simulink model "backtoback_harness"  (R2026b)
settings: Solver=ode4  StopTime=8  FixedStep=0.001
undefined symbols (not defined in the file or in its folder): Dgainphi, Igainphi, Pgainphi, ref_phi
libraries: slpidlib x1
settings Model: Creator=Minh  LastModifiedBy=Minh
settings DataIOCC: SaveTime=off

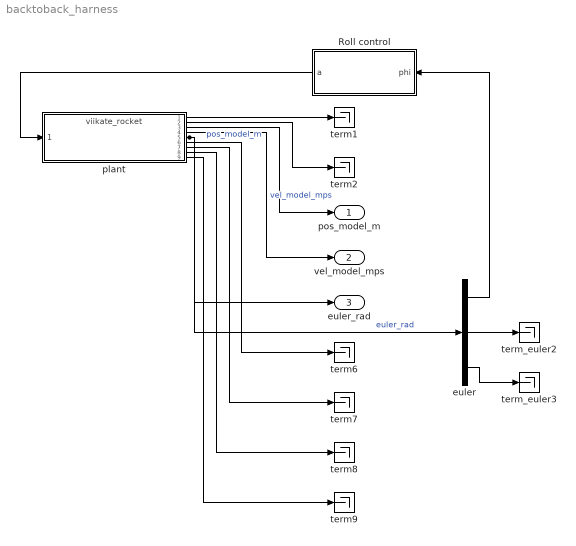
== system backtoback_harness ==
  Roll control : Subsystem
  euler : Demux  Outputs=3
  plant : ModelReference  ModelNameDialog=viikate_rocket  SimulationMode=Normal  ModelReferenceVersion=5.1
  term{1..2,6..9} (6 alike) : Terminator
  term_euler2 : Terminator
  term_euler3 : Terminator
  pos_model_m : Outport
  vel_model_mps : Outport  Port=2
  euler_rad : Outport  Port=3
  wires:
  euler/3 -> term_euler3/1
  euler/2 -> term_euler2/1
  euler/1 -> Roll control/1(phi)
  Roll control/1(a) -> plant/1
  plant/9 -> term9/1
  plant/8 -> term8/1
  plant/7 -> term7/1
  plant/5 -> euler_rad/1, euler/1  "euler_rad"
  plant/4 -> vel_model_mps/1  "vel_model_mps"
  plant/3 -> pos_model_m/1  "pos_model_m"
  plant/6 -> term6/1
  plant/2 -> term2/1
  plant/1 -> term1/1

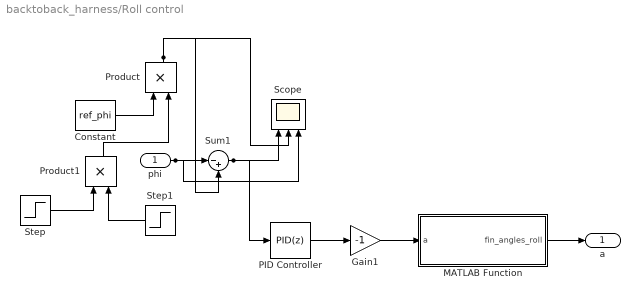
== system backtoback_harness/Roll control ==
  phi : Inport
  Constant : Constant  Value=ref_phi
  Gain1 : Gain  Gain=-1
  MATLAB Function : MATLAB Function  TreatAsAtomicUnit=on
  PID Controller : slpidlib/PID Controller  Controller=PID  Form=Parallel  TimeDomain=Discrete-time  UseExternalTs=off  SampleTime=0.001  IntegratorMethod=Forward Euler  FilterMethod=Forward Euler  ControllerParametersSource=internal  P=Pgainphi  I=Igainphi  UseKiTs=off  D=Dgainphi  UseExternalDerivativeSource=off  N=100  UseFilter=off  TunerSelectOption=Transfer Function Based (PID Tuner App)  InitialConditionSource=internal  InitialConditionForIntegrator=0  InitialConditionForFilter=0  DifferentiatorICPrevScaledInput=0  ExternalReset=none  TrackingMode=off  Kt=1  LimitOutput=on  SatLimitsSource=internal  UpperSaturationLimit=deg2rad(20)  LowerSaturationLimit=-deg2rad(20)  LinearizeAsGain=on  AntiWindupMode=clamping  Kb=1  LimitIntegrator=on  UpperIntegratorSaturationLimit=deg2rad(20)  LowerIntegratorSaturationLimit=-deg2rad(20)  POutMin=[]  POutMax=[]  IOutMin=[]  IOutMax=[]  DOutMin=[]  DOutMax=[]  NOutMin=[]  NOutMax=[]  SumOutMin=[]  SumOutMax=[]  SaturationOutMin=[]  SaturationOutMax=[]  PParamMin=[]  PParamMax=[]  IParamMin=[]  IParamMax=[]  DParamMin=[]  DParamMax=[]  NParamMin=[]  NParamMax=[]  KbParamMin=[]  KbParamMax=[]  KtParamMin=[]  KtParamMax=[]  KbOutMin=[]  KbOutMax=[]  KtOutMin=[]  KtOutMax=[]  IntegratorOutMin=[]  IntegratorOutMax=[]  FilterOutMin=[]  FilterOutMax=[]  SumI1OutMin=[]  SumI1OutMax=[]  SumI2OutMin=[]  SumI2OutMax=[]  SumI3OutMin=[]  SumI3OutMax=[]  SumI4OutMin=[]  SumI4OutMax=[]  SumDOutMin=[]  SumDOutMax=[]  DifferentiatorOutMin=[]  DifferentiatorOutMax=[]  FilterDiffOutCoefMin=[]  FilterDiffOutCoefMax=[]  ReciprocalOutMin=[]  ReciprocalOutMax=[]  SumDenOutMin=[]  SumDenOutMax=[]  SumNumOutMin=[]  SumNumOutMax=[]  DivideOutMin=[]  DivideOutMax=[]  UdiffTsProdOutMin=[]  UdiffTsProdOutMax=[]  NTsProdOutMin=[]  NTsProdOutMax=[]  UintegralTsProdOutMin=[]  UintegralTsProdOutMax=[]  UngainTsProdOutMin=[]  UngainTsProdOutMax=[]  ClampingZeroOutDataTypeStr=Inherit: Inherit via back propagation  ClampingZeroOutMin=[]  ClampingZeroOutMax=[]  FilterDenConstantOutDataTypeStr=Inherit: Inherit via back propagation  FilterDenConstantOutMin=[]  FilterDenConstantOutMax=[]  PCopyOutDataTypeStr=Inherit: Inherit via back propagation  PCopyOutMin=[]  PCopyOutMax=[]  NCopyOutDataTypeStr=Inherit: Inherit via back propagation  NCopyOutMin=[]  NCopyOutMax=[]  IntegratorContinuousStateAttributes=''  IntegratorStateMustResolveToSignalObject=off  IntegratorRTWStateStorageClass=Auto  FilterContinuousStateAttributes=''  FilterStateMustResolveToSignalObject=off  FilterRTWStateStorageClass=Auto  ParallelPVariant=InternalParameters  IdealPVariant=Disabled  IVariant=InternalParameters  DVariant=InternalParameters  IntegratorVariant=Discrete  SatVariant=Enabled  AWVariant=DiscClampingParallel  PCopyVariant=Disabled  TRVariant=Disabled  FdbkBlocksVariant=Forward  IdealPFdbkVariant=Disabled  SatFdbkVariant=Disabled  DerivativeFilterVariant=Differentiator  NVariant=Passthrough  NCopyVariant=Disabled_SignalSpec  FilterICVariant=InternalICsDifferentiator  IntegratorICVariant=InternalICs  ExternalResetVariant=Disabled  TRSumVariant=Passthrough  SumFdbkVariant=Disabled  SumVariant=Sum_PID  TsampFilterVariant=InternalTs  TsampNgainVariant=Passthrough  TsampIntegralVariant=Disabled_SignalSpec  ExternalSaturationOutDataTypeStr=Inherit: Same as second input  DerivativeSourceVariant=ErrorSignal  PreIntVariant=InternalPreInt
  Product : Product
  Product1 : Product
  Scope : Scope  NumInputPorts=3
      settings: ActiveDisplayYMinimum=-3.92695  ActiveDisplayYMaximum=3.92695  DataLoggingVariableName=ScopeData9
  Step : Step  Time=4  InitialValue=1  FinalValue=0  SampleTime=0
  Step1 : Step  Time=2  SampleTime=0
  Sum1 : Sum  Inputs=|-+
  a : Outport  OutMin=[-deg2rad(15)]  OutMax=[deg2rad(15)]
  wires:
  MATLAB Function/1(fin_angles_roll) -> a/1
  Gain1/1 -> MATLAB Function/1(a)
  Sum1/1 -> PID Controller/1, Scope/1
  phi/1 -> Sum1/1, Scope/3
  Product/1 -> Sum1/2, Scope/2
  Step1/1 -> Product1/2
  Product1/1 -> Product/2
  Constant/1 -> Product/1
  PID Controller/1 -> Gain1/1
  Step/1 -> Product1/1

== matlab function backtoback_harness/Roll control/MATLAB Function ==
  data: a input; fin_angles_roll output
function fin_angles_roll = finangles_roll(a)
    fin_angles_roll = [a a a a]';
end
